simulink model "Simulateur_palan_generateur_trajectoire_version2024"  (R2024b)
settings: Solver=FixedStepDiscrete  StartTime=0.0  StopTime=20  RelTol=1e-3
values from neighbouring files (symbols this model uses):
  Ck = [1 0 0 0; 0 0 1 0]    [Script_projet_section2.m]
  F = sysd.A    [Script_projet_section2.m]    (also in labo6_simulation.m)
  G = 0.002    [Essai_boucle_ouverte.mat]    (also in PAR_PAL1_IDENT.m; Script_projet_section2.m = sysd.B; labo6_simulation.m = sysd.B; mncarres_incomplet.m)
  Kr = [0.1 0 0 0]    [Essai_boucle_ouverte.mat]    (also in Script_projet_section2.m = [9.0560    4.5832  -13.7344    0.1]; labo6_simulation.m = [9.9952 2.8361 -8.7562 1.2009])
  L = 0.1    [ETAT_PAL_IDENT.m]    (also in Essai_boucle_ouverte.mat; Script_projet_section2.m = 1; labo6_simulation.m; p1_cre_18V_droite_0m.mat = 0)
  Rf = diag([xres^2*c1 theta_res^2*c2])    [Script_projet_section2.m]
  Tech = '0.0002'    [Essai_boucle_ouverte.mat]    (also in Script_projet_section2.m = 0.0002; labo6_simulation.m = 0.0002; p1_cre_18V_droite_0m.mat = 0.0002; p1_cre_18V_droite_1m.mat = 0.0002)
  xd_ref = 0.5    [Script_projet_section2.m]    (also in labo6_simulation.m)
undefined symbols (not defined in the file or in its folder): Discrete, Time
libraries: cstblocks x2, simulink x2, ctrlSharedLib x1
settings Model: Creator=Ale  LastModifiedBy=Ale

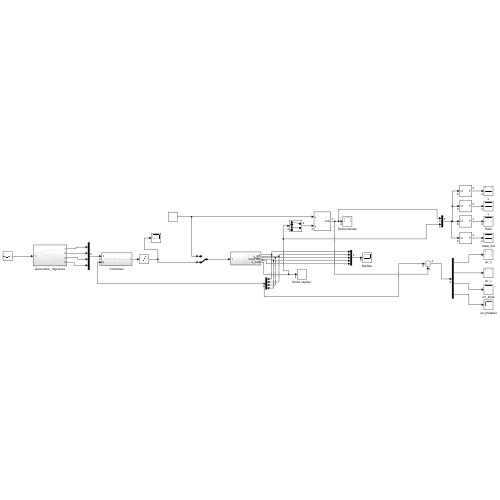
[thumbnail: Simulink's stored preview of the top-level diagram]
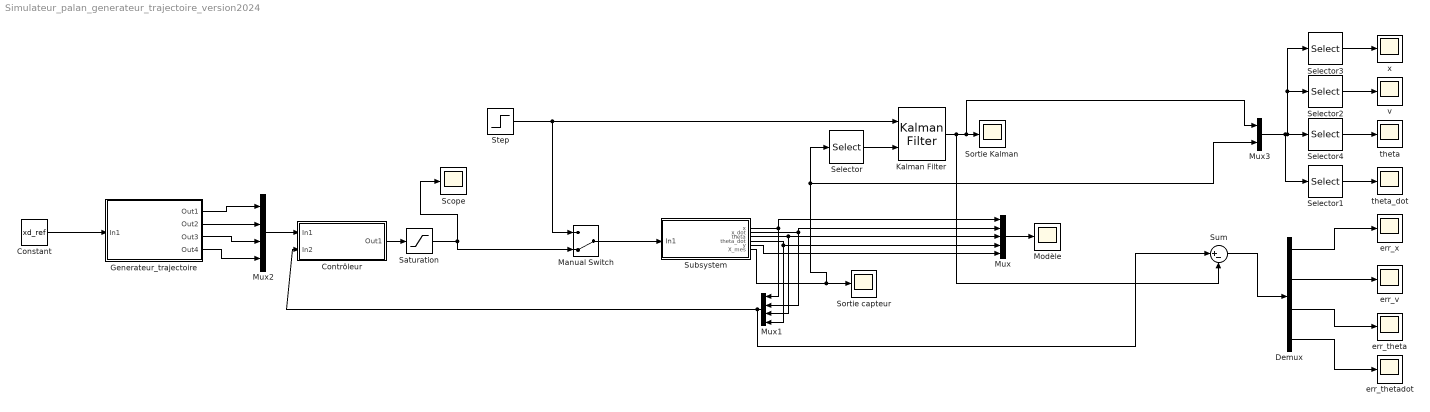
== system Simulateur_palan_generateur_trajectoire_version2024 ==
  Constant : Constant  Value=xd_ref
  Contrôleur : Subsystem
  Demux : Demux
  Generateur_trajectoire : Subsystem
  Kalman Filter : ctrlSharedLib/Kalman Filter  TimeDomain=Discrete-Time  UseCurrentEstimator=on  ModelSource=Individual A, B, C, D matrices  ModelSourceVariable=ss(0.95,1,1,0,1)  A=F  B=G  C=Ck  D=0  NumberOfStates=1  NumberOfInputs=1  NumberOfOutputs=1  InitialEstimateSource=Dialog  X0=0  P0=10  UseK=off  UseGH=off  NumberOfProcessNoiseInputs=1  G=1  TimeInvariantG=on  H=0  TimeInvariantH=on  Q=Qf  TimeInvariantQ=on  R=Rf  TimeInvariantR=on  N=0  TimeInvariantN=on  AddInputPort=on  AddEnablePort=off  OutputEstimatedY=off  OutputP=off  Ts=-1
  Manual Switch : ManualSwitch  CurrentSetting=0
  Modèle : Scope
  Mux : Mux  Inputs=5
  Mux1 : Mux
  Mux2 : Mux
  Mux3 : Mux  Inputs=2
  Saturation : Saturate  UpperLimit=24  LowerLimit=-24
  Scope : Scope
  Selector : Selector  InputPortWidth=4  IndexOptions=Index vector (dialog)  Indices=[1 3]  OutputSizes=1
  Selector1 : Selector  InputPortWidth=8  IndexOptions=Index vector (dialog)  Indices=[4 8]  OutputSizes=1
  Selector2 : Selector  InputPortWidth=8  IndexOptions=Index vector (dialog)  Indices=[2 6]  OutputSizes=1
  Selector3 : Selector  InputPortWidth=8  IndexOptions=Index vector (dialog)  Indices=[1 5]  OutputSizes=1
  Selector4 : Selector  InputPortWidth=8  IndexOptions=Index vector (dialog)  Indices=[3 7]  OutputSizes=1
  Sortie Kalman : Scope
  Sortie capteur : Scope
  Step : Step  After=19.92  SampleTime=Tech
  Subsystem : Subsystem
  Sum : Sum  Inputs=|+-
  err_theta : Scope
  err_thetadot : Scope
  err_v : Scope
  err_x : Scope
  theta : Scope
  theta_dot : Scope
  v : Scope
  x : Scope
  wires:
  Subsystem/1(x) -> Mux/1, Mux1/1
  Subsystem/2(x_dot) -> Mux/2, Mux1/2
  Subsystem/3(theta) -> Mux1/3, Mux/3
  Subsystem/4(theta_dot) -> Mux1/4, Mux/4
  Subsystem/5(y) -> Mux/5
  Mux/1 -> Modèle/1
  Mux1/1 -> Sum/1, Contrôleur/2(In2)
  Contrôleur/1(Out1) -> Saturation/1
  Saturation/1 -> Manual Switch/2, Scope/1
  Mux2/1 -> Contrôleur/1(In1)
  Generateur_trajectoire/1(Out1) -> Mux2/1
  Generateur_trajectoire/2(Out2) -> Mux2/2
  Generateur_trajectoire/3(Out3) -> Mux2/3
  Generateur_trajectoire/4(Out4) -> Mux2/4
  Constant/1 -> Generateur_trajectoire/1(In1)
  Subsystem/6(X_mes) -> Mux3/2, Selector/1, Sortie capteur/1
  Step/1 -> Manual Switch/1, Kalman Filter/1
  Manual Switch/1 -> Subsystem/1(In1)
  Kalman Filter/1 -> Mux3/1, Sortie Kalman/1, Sum/2
  Selector/1 -> Kalman Filter/2
  Mux3/1 -> Selector3/1, Selector2/1, Selector4/1, Selector1/1
  Selector1/1 -> theta_dot/1
  Selector3/1 -> x/1
  Selector2/1 -> v/1
  Selector4/1 -> theta/1
  Sum/1 -> Demux/1
  Demux/1 -> err_x/1
  Demux/4 -> err_thetadot/1
  Demux/3 -> err_theta/1
  Demux/2 -> err_v/1

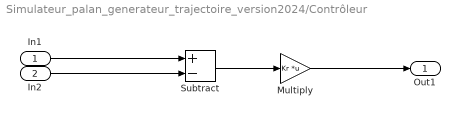
== system Simulateur_palan_generateur_trajectoire_version2024/Contrôleur ==
  In1 : Inport
  In2 : Inport  Port=2
  Multiply : Gain  Gain=Kr  Multiplication=Matrix(K*u)
  Subtract : Sum  Inputs=+-
  Out1 : Outport
  wires:
  In1/1 -> Subtract/1
  In2/1 -> Subtract/2
  Subtract/1 -> Multiply/1
  Multiply/1 -> Out1/1

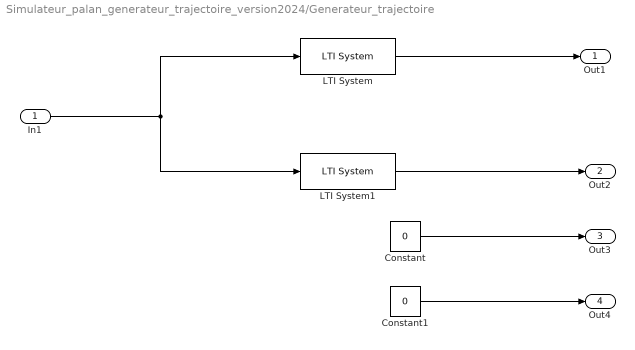
== system Simulateur_palan_generateur_trajectoire_version2024/Generateur_trajectoire ==
  In1 : Inport
  Constant : Constant  Value=0
  Constant1 : Constant  Value=0
  LTI System : cstblocks/LTI System  sys=H_pos_d  IC=[]  PadeOrder=0
  LTI System1 : cstblocks/LTI System  sys=H_vit_d  IC=[]  PadeOrder=0
  Out1 : Outport
  Out2 : Outport  Port=2
  Out3 : Outport  Port=3
  Out4 : Outport  Port=4
  wires:
  In1/1 -> LTI System/1, LTI System1/1
  LTI System/1 -> Out1/1
  LTI System1/1 -> Out2/1
  Constant/1 -> Out3/1
  Constant1/1 -> Out4/1

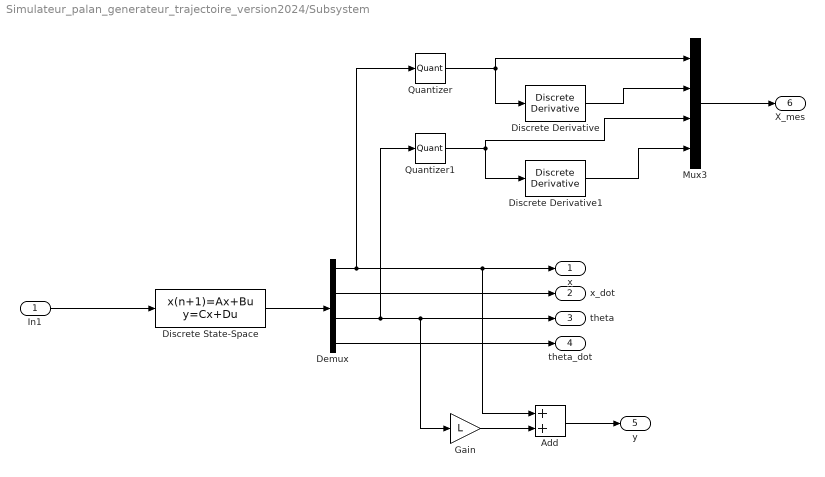
== system Simulateur_palan_generateur_trajectoire_version2024/Subsystem ==
  In1 : Inport
  Add : Sum
  Demux : Demux
  Discrete Derivative : simulink/Discrete/Discrete Derivative  gainval=1.0  ICPrevScaledInput=0.0  OutMin=[]  OutMax=[]  OutDataType=fixdt(1, 16)  OutScaling=2^-10  DoSatur=off
  Discrete Derivative1 : simulink/Discrete/Discrete Derivative  gainval=1.0  ICPrevScaledInput=0.0  OutMin=[]  OutMax=[]  OutDataType=fixdt(1, 16)  OutScaling=2^-10  DoSatur=off
  Discrete State-Space : DiscreteStateSpace  A=F  B=G  C=[1 0 0 0;0 1 0 0; 0 0 1 0; 0 0 0 1]  D=[0;0;0;0]  SampleTime=-1
  Gain : Gain  Gain=L
  Mux3 : Mux
  Quantizer : Quantizer  QuantizationInterval=xres
  Quantizer1 : Quantizer  QuantizationInterval=theta_res
  x : Outport
  x_dot : Outport  Port=2
  theta : Outport  Port=3
  theta_dot : Outport  Port=4
  y : Outport  Port=5
  X_mes : Outport  Port=6
  wires:
  Demux/2 -> x_dot/1
  Demux/1 -> Quantizer/1, x/1, Add/1
  Demux/4 -> theta_dot/1
  Demux/3 -> Quantizer1/1, theta/1, Gain/1
  Gain/1 -> Add/2
  Add/1 -> y/1
  In1/1 -> Discrete State-Space/1
  Discrete State-Space/1 -> Demux/1
  Quantizer/1 -> Discrete Derivative/1, Mux3/1
  Discrete Derivative/1 -> Mux3/2
  Quantizer1/1 -> Mux3/3, Discrete Derivative1/1
  Discrete Derivative1/1 -> Mux3/4
  Mux3/1 -> X_mes/1
